simulink model "Complete_SAD_model"  (R2025b)
settings: Solver=ode4  StartTime=0.0  StopTime=10  FixedStep=0.01  RelTol=1e-3
values from neighbouring files (symbols this model uses):
  A = eye(3)    [Initial_condition.m]
  a_pink = exp(-2*pi*fc_pink*Ts_m*k_pink)    [Initial_condition.m]
  acc = deg2rad(0.5*randn)    [Initial_condition.m]
  Ap = eye(3)    [Initial_condition.m]
  D = 500*10^-12    (= 5e-10)    [Initial_condition.m]
  delay = 1    [Initial_condition.m]
  inv_Ir = inv(Ir)    [Initial_condition.m]
  Ir = diag([Irx,Iry,Irz])    [Initial_condition.m]
  J_B = diag([Ix,Iy,Iz])    [Initial_condition.m]
  m = [0.01; 0.01; 0.01]    [Initial_condition.m]
  m_max = [0.65; 0.65; 0.5]    [Initial_condition.m]
  Mr_max = [0.01; 0.01; 0.01]    [Initial_condition.m]
  mu_earth = 398600.433    [Initial_condition.m]
  mu_sun = 132712440017.987    (= 132712440018)    [Initial_condition.m]
  non_ort = deg2rad(-1+2*rand)    [Initial_condition.m]
  omega0 = [wx;wy;wz]    [Initial_condition.m]
  rES0_ECI = [0 AU 0]    [Initial_condition.m]
  seed = 0    [Initial_condition.m]
  sigma = (2*pi/60)/3    (= 0.0349065850399)    [Initial_condition.m]
  Ts_m = 1/f_m    (= 0.1)    [Initial_condition.m]
  Ts_ss = 1/f_ss    (= 0.1)    [Initial_condition.m]
  vES0_ECI = [(-sqrt(mu_sun/norm(rES0_ECI))) 0 0 ]    [Initial_condition.m]
  w_max = [250; 250; 250]    [Initial_condition.m]
undefined symbols (not defined in the file or in its folder): dspblkCoreblockFVToolHelper, gcbh, K, r0_ECI, v0_ECI
libraries: matrix_library x15, dspmathops x3, dspfdesign x3, vrlib x2
(part 3 of 3)

== matlab function Complete_SAD_model/Subsystem3/Disturbance Torques/MAGNETIC FIELD PERTURBATION1/MATLAB Function ==
  data: alfa input; delta input; r_scalar input; B_IN output; t input
function B_IN = fcn(alfa, delta, r_scalar, t)
% Magnetic field model of order 5 with g and h coefficients updated to 2025
% The output B_IN is in nT

alfa0_G = 0; % We assume the rigt ascension of Greenwich is zero at t=0
alfa_G = (2*pi/86164)*t + alfa0_G; % Right ascension of Greenwich as a function of time

%% Components of B wrt the Earth rotating fixed frame
%Br = @(psi,r,theta)1.0./r.^6.*(cos(theta).^2.*(-3.355125e+3)+cos(theta).^4.*3.9143125e+3+((sqrt(1.0e+1).*sin(theta.*2.0))./1.6e+1+sqrt(1.0e+1).*sin(theta.*4.0).*(7.0./3.2e+1)).*(cos(psi).*7.996e+2+sin(psi).*2.786e+2)+(sqrt(3.5e+1).*sin(theta).^4.*(cos(psi.*4.0).*1.2e+1-sin(psi.*4.0).*3.754e+2))./8.0-(sqrt(7.0e+1).*cos(theta).*sin(theta).^3.*(cos(psi.*3.0).*2.811e+2-sin(psi.*3.0).*2.12e+2))./4.0-(sqrt(5.0).*sin(theta).^2.*(sin(theta).^2.*7.0-6.0).*(cos(psi.*2.0).*(2.79e+2./5.0)-sin(psi.*2.0).*1.34e+2))./4.0+3.355125e+2).*3.343610149269505e+23+1.0./r.^5.*(cos(theta).*(cos(theta).^2.*5.0-3.0).*6.8045e+2+(sqrt(1.0e+1).*sin(theta).^3.*(cos(psi.*3.0).*4.534e+2-sin(psi.*3.0).*5.496e+2))./4.0+(sqrt(6.0).*sin(theta).*(sin(theta).^2.*5.0-4.0).*(cos(psi).*2.4042e+3+sin(psi).*(5.69e+2./1.0e+1)))./4.0-(sqrt(1.5e+1).*cos(theta).*(cos(psi.*2.0).*1.2438e+3+sin(psi.*2.0).*2.376e+2).*(cos(theta).^2-1.0))./2.0).*4.198537308767232e+19+1.0./r.^4.*(cos(theta).^2.*(-3.8343e+3)+(sqrt(3.0).*sin(theta).^2.*(cos(psi.*2.0).*1.6487e+3-sin(psi.*2.0).*8.142e+2))./2.0+(sqrt(3.0).*sin(theta.*2.0).*(cos(psi).*2.9509e+3-sin(psi).*3.1336e+3))./2.0+1.2781e+3).*4.942556869526643e+15+1.0./r.^7.*(sin(theta).^5.*(cos(psi.*5.0).*(2.09e+2./1.0e+1)+sin(psi.*5.0).*(5.31e+2./5.0)).*7.01560760020114e-1-cos(theta).*(cos(theta).^2.*-7.0e+1+cos(theta).^4.*6.3e+1+1.5e+1).*2.91125e+1-cos(theta).*sin(theta).^4.*(cos(psi.*4.0).*1.419e+2-sin(psi.*4.0).*(4.29e+2./1.0e+1)).*2.218529918662356+sqrt(1.5e+1).*(cos(psi).*3.69e+2+sin(psi).*(4.53e+2./1.0e+1)).*(sin(theta)-sin(theta).^3.*(7.0./2.0)+sin(theta).^5.*(2.1e+1./8.0))+(sqrt(7.0e+1).*sin(theta).^3.*(sin(theta).^2.*9.0-8.0).*(cos(psi.*3.0).*1.387e+2+sin(psi.*3.0).*1.229e+2))./1.6e+1-(sqrt(1.05e+2).*cos(theta).*(cos(psi.*2.0).*(9.36e+2./5.0)+sin(psi.*2.0).*2.2e+2).*(cos(theta).^2.*-4.0+cos(theta).^4.*3.0+1.0))./4.0).*2.556256831319522e+27-1.0./r.^3.*(cos(theta).*2.935e+4+sin(theta).*(cos(psi).*1.4103e+3-sin(psi).*4.5455e+3)).*5.17193205622e+11;
%Btheta = @(psi,r,theta)-(1.0./r.^5.*(cos(theta).*sin(theta).*6.71025e+3-cos(theta).^3.*sin(theta).*1.565725e+4+((sqrt(1.0e+1).*cos(theta.*2.0))./8.0+sqrt(1.0e+1).*cos(theta.*4.0).*(7.0./8.0)).*(cos(psi).*7.996e+2+sin(psi).*2.786e+2)+(sqrt(7.0e+1).*sin(theta).^4.*(cos(psi.*3.0).*2.811e+2-sin(psi.*3.0).*2.12e+2))./4.0-sqrt(5.0).*cos(theta).*sin(theta).^3.*(cos(psi.*2.0).*(2.79e+2./5.0)-sin(psi.*2.0).*1.34e+2).*(7.0./2.0)+(sqrt(3.5e+1).*cos(theta).*sin(theta).^3.*(cos(psi.*4.0).*1.2e+1-sin(psi.*4.0).*3.754e+2))./2.0-sqrt(7.0e+1).*cos(theta).^2.*sin(theta).^2.*(cos(psi.*3.0).*2.811e+2-sin(psi.*3.0).*2.12e+2).*(3.0./4.0)-(sqrt(5.0).*cos(theta).*sin(theta).*(sin(theta).^2.*7.0-6.0).*(cos(psi.*2.0).*(2.79e+2./5.0)-sin(psi.*2.0).*1.34e+2))./2.0).*6.687220298539009e+22+1.0./r.^4.*(sin(theta).*(cos(theta).^2.*5.0-3.0).*(-6.8045e+2)-cos(theta).^2.*sin(theta).*6.8045e+3+sqrt(1.0e+1).*cos(theta).*sin(theta).^2.*(cos(psi.*3.0).*4.534e+2-sin(psi.*3.0).*5.496e+2).*(3.0./4.0)+sqrt(1.5e+1).*cos(theta).^2.*sin(theta).*(cos(psi.*2.0).*1.2438e+3+sin(psi.*2.0).*2.376e+2)+(sqrt(6.0).*cos(theta).*(sin(theta).^2.*5.0-4.0).*(cos(psi).*2.4042e+3+sin(psi).*(5.69e+2./1.0e+1)))./4.0+sqrt(6.0).*cos(theta).*sin(theta).^2.*(cos(psi).*2.4042e+3+sin(psi).*(5.69e+2./1.0e+1)).*(5.0./2.0)+(sqrt(1.5e+1).*sin(theta).*(cos(psi.*2.0).*1.2438e+3+sin(psi.*2.0).*2.376e+2).*(cos(theta).^2-1.0))./2.0).*1.049634327191808e+19+1.0./r.^3.*(cos(theta).*sin(theta).*7.6686e+3+sqrt(3.0).*cos(theta.*2.0).*(cos(psi).*2.9509e+3-sin(psi).*3.1336e+3)+sqrt(3.0).*cos(theta).*sin(theta).*(cos(psi.*2.0).*1.6487e+3-sin(psi.*2.0).*8.142e+2)).*1.647518956508881e+15+1.0./r.^6.*(cos(theta).*(cos(theta).*sin(theta).*1.4e+2-cos(theta).^3.*sin(theta).*2.52e+2).*(-2.91125e+1)+sin(theta).^5.*(cos(psi.*4.0).*1.419e+2-sin(psi.*4.0).*(4.29e+2./1.0e+1)).*2.218529918662356+sin(theta).*(cos(theta).^2.*-7.0e+1+cos(theta).^4.*6.3e+1+1.5e+1).*2.91125e+1+cos(theta).*sin(theta).^4.*(cos(psi.*5.0).*(2.09e+2./1.0e+1)+sin(psi.*5.0).*(5.31e+2./5.0)).*3.50780380010057-cos(theta).^2.*sin(theta).^3.*(cos(psi.*4.0).*1.419e+2-sin(psi.*4.0).*(4.29e+2./1.0e+1)).*8.874119674649425+sqrt(1.5e+1).*(cos(psi).*3.69e+2+sin(psi).*(4.53e+2./1.0e+1)).*(cos(theta)-cos(theta).*sin(theta).^2.*(2.1e+1./2.0)+cos(theta).*sin(theta).^4.*(1.05e+2./8.0))-(sqrt(1.05e+2).*cos(theta).*(cos(psi.*2.0).*(9.36e+2./5.0)+sin(psi.*2.0).*2.2e+2).*(cos(theta).*sin(theta).*8.0-cos(theta).^3.*sin(theta).*1.2e+1))./4.0+sqrt(7.0e+1).*cos(theta).*sin(theta).^4.*(cos(psi.*3.0).*1.387e+2+sin(psi.*3.0).*1.229e+2).*(9.0./8.0)+(sqrt(1.05e+2).*sin(theta).*(cos(psi.*2.0).*(9.36e+2./5.0)+sin(psi.*2.0).*2.2e+2).*(cos(theta).^2.*-4.0+cos(theta).^4.*3.0+1.0))./4.0+sqrt(7.0e+1).*cos(theta).*sin(theta).^2.*(sin(theta).^2.*9.0-8.0).*(cos(psi.*3.0).*1.387e+2+sin(psi.*3.0).*1.229e+2).*(3.0./1.6e+1)).*4.260428052199203e+26+1.0./r.^2.*(sin(theta).*2.935e+4-cos(theta).*(cos(psi).*1.4103e+3-sin(psi).*4.5455e+3)).*2.58596602811e+11)./r;
%Bpsi = @(psi,r,theta)-(1.0./r.^3.*((sqrt(3.0).*sin(theta).^2.*(cos(psi.*2.0).*1.6284e+3+sin(psi.*2.0).*3.2974e+3))./2.0+(sqrt(3.0).*sin(theta.*2.0).*(cos(psi).*3.1336e+3+sin(psi).*2.9509e+3))./2.0).*-1.647518956508881e+15-1.0./r.^4.*((sqrt(1.0e+1).*sin(theta).^3.*(cos(psi.*3.0).*1.6488e+3+sin(psi.*3.0).*1.3602e+3))./4.0-(sqrt(6.0).*sin(theta).*(sin(theta).^2.*5.0-4.0).*(cos(psi).*(5.69e+2./1.0e+1)-sin(psi).*2.4042e+3))./4.0+(sqrt(1.5e+1).*cos(theta).*(cos(psi.*2.0).*4.752e+2-sin(psi.*2.0).*2.4876e+3).*(cos(theta).^2-1.0))./2.0).*1.049634327191808e+19+1.0./r.^5.*(((sqrt(1.0e+1).*sin(theta.*2.0))./1.6e+1+sqrt(1.0e+1).*sin(theta.*4.0).*(7.0./3.2e+1)).*(cos(psi).*2.786e+2-sin(psi).*7.996e+2)-(sqrt(3.5e+1).*sin(theta).^4.*(cos(psi.*4.0).*1.5016e+3+sin(psi.*4.0).*4.8e+1))./8.0+(sqrt(7.0e+1).*cos(theta).*sin(theta).^3.*(cos(psi.*3.0).*6.36e+2+sin(psi.*3.0).*8.433e+2))./4.0+(sqrt(5.0).*sin(theta).^2.*(sin(theta).^2.*7.0-6.0).*(cos(psi.*2.0).*2.68e+2+sin(psi.*2.0).*(5.58e+2./5.0)))./4.0).*6.687220298539009e+22+1.0./r.^6.*(sin(theta).^5.*(cos(psi.*5.0).*5.31e+2-sin(psi.*5.0).*(2.09e+2./2.0)).*7.01560760020114e-1+cos(theta).*sin(theta).^4.*(cos(psi.*4.0).*(8.58e+2./5.0)+sin(psi.*4.0).*5.676e+2).*2.218529918662356+sqrt(1.5e+1).*(cos(psi).*(4.53e+2./1.0e+1)-sin(psi).*3.69e+2).*(sin(theta)-sin(theta).^3.*(7.0./2.0)+sin(theta).^5.*(2.1e+1./8.0))+(sqrt(7.0e+1).*sin(theta).^3.*(sin(theta).^2.*9.0-8.0).*(cos(psi.*3.0).*3.687e+2-sin(psi.*3.0).*4.161e+2))./1.6e+1-(sqrt(1.05e+2).*cos(theta).*(cos(psi.*2.0).*4.4e+2-sin(psi.*2.0).*3.744e+2).*(cos(theta).^2.*-4.0+cos(theta).^4.*3.0+1.0))./4.0).*4.260428052199203e+26+1.0./r.^2.*sin(theta).*(cos(psi).*4.5455e+3+sin(psi).*1.4103e+3).*2.58596602811e+11)./(r.*sin(theta));
Br = @(psi,r,theta)1.0./r.^6.*(cos(theta).^2.*(-3.355125e+3)+cos(theta).^4.*3.9143125e+3+((sqrt(1.0e+1).*sin(theta.*2.0))./1.6e+1+sqrt(1.0e+1).*sin(theta.*4.0).*(7.0./3.2e+1)).*(cos(psi).*7.996e+2+sin(psi).*2.786e+2)+(sqrt(3.5e+1).*sin(theta).^4.*(cos(psi.*4.0).*1.2e+1-sin(psi.*4.0).*3.754e+2))./8.0-(sqrt(7.0e+1).*cos(theta).*sin(theta).^3.*(cos(psi.*3.0).*2.811e+2-sin(psi.*3.0).*2.12e+2))./4.0-(sqrt(5.0).*sin(theta).^2.*(sin(theta).^2.*7.0-6.0).*(cos(psi.*2.0).*(2.79e+2./5.0)-sin(psi.*2.0).*1.34e+2))./4.0+3.355125e+2).*3.343610149269505e+23+1.0./r.^8.*(cos(theta).^2.*4.2196875e+2-cos(theta).^4.*1.26590625e+3+cos(theta).^6.*9.2833125e+2-sin(theta).^6.*(cos(psi.*6.0).*(3.04e+2./5.0)-sin(psi.*6.0).*(3.64e+2./5.0)).*6.716932893813961e-1+(cos(psi).*(3.19e+2./5.0)-sin(psi).*(9.2e+1./5.0)).*(sqrt(2.1e+1).*sin(theta.*2.0).*(5.0./2.56e+2)+sqrt(2.1e+1).*sin(theta.*4.0).*(3.0./6.4e+1)+sqrt(2.1e+1).*sin(theta.*6.0).*(3.3e+1./2.56e+2))+cos(theta).*sin(theta).^5.*(cos(psi.*5.0).*(1.49e+2./1.0e+1)+sin(psi.*5.0).*(1.09e+2./1.0e+1)).*2.326813808623286+sin(theta).^4.*(sin(theta).^2.*1.1e+1-1.0e+1).*(cos(psi.*4.0).*(4.09e+2./1.0e+1)+sin(psi.*4.0).*(2.99e+2./5.0)).*4.960783708246107e-1+(sqrt(2.1e+2).*sin(theta).^2.*(cos(psi.*2.0).*(7.67e+2./1.0e+1)+sin(psi.*2.0).*(8.4e+1./5.0)).*(sin(theta).^2.*-4.8e+1+sin(theta).^4.*3.3e+1+1.6e+1))./3.2e+1-(sqrt(2.1e+2).*cos(theta).*sin(theta).^3.*(cos(psi.*3.0).*1.157e+2-sin(psi.*3.0).*(4.89e+2./1.0e+1)).*(cos(theta).^2.*1.1e+1-3.0))./1.6e+1-6.43e+2./3.2e+1).*1.900023098439278e+31+1.0./r.^10.*((cos(psi).*(1.09e+2./1.0e+1)+sin(psi).*(3.6e+1./5.0)).*(sin(theta.*2.0).*5.126953125e-2+sin(theta.*4.0).*1.1279296875e-1+sin(theta.*6.0).*2.0947265625e-1+sin(theta.*8.0).*5.23681640625e-1)-cos(theta).^2.*2.27390625e+2+cos(theta).^4.*1.2506484375e+3-cos(theta).^6.*2.167790625e+3+cos(theta).^8.*1.16131640625e+3+sin(theta).^8.*(cos(psi.*8.0)+sin(psi.*8.0).*(3.9e+1./1.0e+1)).*6.267066542400439e-1-cos(theta).*sin(theta).^7.*(cos(psi.*7.0).*(8.4e+1./5.0)+sin(psi.*7.0).*(2.6e+1./5.0)).*2.506826616960176-sin(theta).^6.*(sin(theta).^2.*1.5e+1-1.4e+1).*(cos(psi.*6.0).*(1.49e+2./1.0e+1)+sin(psi.*6.0).*(7.0./1.0e+1)).*4.576818286211503e-1-sin(theta).^4.*(cos(psi.*4.0).*(1.09e+2./5.0)+sin(psi.*4.0).*(9.7e+1./1.0e+1)).*(sin(theta).^2.*-1.04e+2+sin(theta).^4.*6.5e+1+4.0e+1).*4.113264556590057e-1+cos(theta).*sin(theta).^5.*(cos(psi.*5.0).*(1.69e+2./1.0e+1)+sin(psi.*5.0).*(1.27e+2./1.0e+1)).*(cos(theta).^2.*5.0-1.0).*2.96611725366682+cos(theta).*sin(theta).^3.*(cos(psi.*3.0).*2.0+sin(psi.*3.0).*(2.3e+1./2.0)).*(cos(theta).^2.*-2.6e+1+cos(theta).^4.*3.9e+1+3.0).*1.062040341747902+sqrt(7.0e+1).*sin(theta).^2.*(cos(psi.*2.0).*(3.5e+1./2.0)+sin(psi.*2.0).*(6.3e+1./5.0)).*(sin(theta).^2.*1.76e+2-sin(theta).^4.*2.86e+2+sin(theta).^6.*1.43e+2-3.2e+1).*4.6875e-2+6.31640625).*9.915589987374597e+38-1.0./r.^11.*(sin(theta).^9.*(cos(psi.*9.0).*(6.4e+1./5.0)-sin(psi.*9.0).*(4.9e+1./5.0)).*6.090493921755238e-1-cos(theta).*(cos(theta).^2.*-4.62e+3+cos(theta).^4.*1.8018e+4-cos(theta).^6.*2.574e+4+cos(theta).^8.*1.2155e+4+3.15e+2).*3.671875e-2+cos(theta).*sin(theta).^8.*(cos(psi.*8.0).*(8.7e+1./1.0e+1)-sin(psi.*8.0).*(4.0./5.0)).*2.583977731709148+sin(theta).^7.*(sin(theta).^2.*1.7e+1-1.6e+1).*(cos(psi.*7.0).*(4.3e+1./5.0)-sin(psi.*7.0).*(3.0./5.0)).*4.431485250278681e-1-sin(theta).^3.*(cos(psi.*3.0)./5.0-sin(psi.*3.0).*(8.3e+1./1.0e+1)).*(sin(theta).^2.*3.12e+2-sin(theta).^4.*4.68e+2+sin(theta).^6.*2.21e+2-6.4e+1).*3.754879637718099e-1+sin(theta).^5.*(cos(psi.*5.0).*(1.31e+2./1.0e+1)+sin(psi.*5.0).*(5.3e+1./1.0e+1)).*(sin(theta).^2.*-1.4e+2+sin(theta).^4.*8.5e+1+5.6e+1).*3.96364090436432e-1-cos(theta).*sin(theta).^6.*(cos(psi.*6.0).*(1.2e+1./5.0)+sin(psi.*6.0).*(3.6e+1./5.0)).*(cos(theta).^2.*1.7e+1-3.0).*1.023407680863301-sqrt(5.0).*sin(theta).*(cos(psi).*8.0-sin(psi).*(1.24e+2./5.0)).*(sin(theta).^2.*-1.408e+3+sin(theta).^4.*4.576e+3-sin(theta).^6.*5.72e+3+sin(theta).^8.*2.431e+3+1.28e+2).*2.34375e-2+cos(theta).*sin(theta).^4.*(cos(psi.*4.0).*(5.0./2.0)+sin(psi.*4.0).*(1.7e+1./5.0)).*(cos(theta).^2.*-1.0e+1+cos(theta).^4.*1.7e+1+1.0).*3.316219904216999+sqrt(1.1e+2).*cos(theta).*(cos(psi.*2.0).*3.0+sin(psi.*2.0).*(1.21e+2./1.0e+1)).*(cos(theta).^2.*-9.8e+1+cos(theta).^4.*3.64e+2-cos(theta).^6.*4.94e+2+cos(theta).^8.*2.21e+2+7.0).*4.6875e-2).*7.019135978840395e+42+1.0./r.^5.*(cos(theta).*(cos(theta).^2.*5.0-3.0).*6.8045e+2+(sqrt(1.0e+1).*sin(theta).^3.*(cos(psi.*3.0).*4.534e+2-sin(psi.*3.0).*5.496e+2))./4.0+(sqrt(6.0).*sin(theta).*(sin(theta).^2.*5.0-4.0).*(cos(psi).*2.4042e+3+sin(psi).*(5.69e+2./1.0e+1)))./4.0-(sqrt(1.5e+1).*cos(theta).*(cos(psi.*2.0).*1.2438e+3+sin(psi.*2.0).*2.376e+2).*(cos(theta).^2-1.0))./2.0).*4.198537308767232e+19+1.0./r.^4.*(cos(theta).^2.*(-3.8343e+3)+(sqrt(3.0).*sin(theta).^2.*(cos(psi.*2.0).*1.6487e+3-sin(psi.*2.0).*8.142e+2))./2.0+(sqrt(3.0).*sin(theta.*2.0).*(cos(psi).*2.9509e+3-sin(psi).*3.1336e+3))./2.0+1.2781e+3).*4.942556869526643e+15+1.0./r.^9.*(sin(theta).^7.*(cos(psi.*7.0).*(1.43e+2./1.0e+1)-sin(psi.*7.0).*(1.1e+1./5.0)).*6.472598492877493e-1+cos(theta).*(cos(theta).^2.*3.15e+2-cos(theta).^4.*6.93e+2+cos(theta).^6.*4.29e+2-3.5e+1).*4.975-cos(theta).*sin(theta).^6.*(cos(psi.*6.0).*(5.6e+1./5.0)+sin(psi.*6.0).*(2.51e+2./1.0e+1)).*2.421824596249695-sin(theta).^5.*(sin(theta).^2.*1.3e+1-1.2e+1).*(cos(psi.*5.0).*(5.0./2.0)-sin(psi.*5.0).*(3.7e+1./5.0)).*4.749588797990833e-1+cos(theta).*sin(theta).^4.*(cos(psi.*4.0).*(7.9e+1./5.0)+sin(psi.*4.0).*(4.7e+1./2.0)).*(cos(theta).^2.*1.3e+1-3.0).*9.499177595981665e-1+sqrt(2.1e+1).*sin(theta).^3.*(cos(psi.*3.0).*(5.93e+2./1.0e+1)-sin(psi.*3.0)).*(sin(theta).^2.*-2.2e+2+sin(theta).^4.*1.43e+2+8.0e+1).*3.125e-2+sqrt(4.2e+1).*cos(theta).*(cos(psi.*2.0).*(4.4e+1./5.0)+sin(psi.*2.0).*(7.2e+1./5.0)).*(cos(theta).^2.*1.25e+2-cos(theta).^4.*2.53e+2+cos(theta).^6.*1.43e+2-1.5e+1).*3.125e-2+sqrt(7.0).*sin(theta).*(cos(psi).*(7.69e+2./1.0e+1)+sin(psi).*(4.89e+2./1.0e+1)).*(sin(theta).^2.*4.32e+2-sin(theta).^4.*7.92e+2+sin(theta).^6.*4.29e+2-6.4e+1).*3.125e-2).*1.383433961160759e+35+1.0./r.^7.*(sin(theta).^5.*(cos(psi.*5.0).*(2.09e+2./1.0e+1)+sin(psi.*5.0).*(5.31e+2./5.0)).*7.01560760020114e-1-cos(theta).*(cos(theta).^2.*-7.0e+1+cos(theta).^4.*6.3e+1+1.5e+1).*2.91125e+1-cos(theta).*sin(theta).^4.*(cos(psi.*4.0).*1.419e+2-sin(psi.*4.0).*(4.29e+2./1.0e+1)).*2.218529918662356+sqrt(1.5e+1).*(cos(psi).*3.69e+2+sin(psi).*(4.53e+2./1.0e+1)).*(sin(theta)-sin(theta).^3.*(7.0./2.0)+sin(theta).^5.*(2.1e+1./8.0))+(sqrt(7.0e+1).*sin(theta).^3.*(sin(theta).^2.*9.0-8.0).*(cos(psi.*3.0).*1.387e+2+sin(psi.*3.0).*1.229e+2))./1.6e+1-(sqrt(1.05e+2).*cos(theta).*(cos(psi.*2.0).*(9.36e+2./5.0)+sin(psi.*2.0).*2.2e+2).*(cos(theta).^2.*-4.0+cos(theta).^4.*3.0+1.0))./4.0).*2.556256831319522e+27-1.0./r.^12.*(cos(theta).^2.*1.7595703125e+1-cos(theta).^4.*1.5249609375e+2+cos(theta).^6.*4.5748828125e+2-cos(theta).^8.*5.55521484375e+2+cos(theta).^10.*2.34553515625e+2+sin(theta).^10.*(cos(psi.*1.0e+1).*(3.9e+1./1.0e+1)+sin(psi.*1.0e+1).*9.0).*5.936279171365732e-1+cos(theta).*sin(theta).^9.*(cos(psi.*9.0).*(1.3e+1./5.0)-sin(psi.*9.0).*(9.0./1.0e+1)).*2.65478475211798-sin(theta).^4.*(cos(psi.*4.0)-sin(psi.*4.0).*(2.7e+1./5.0)).*(sin(theta).^2.*5.04e+2-sin(theta).^4.*7.14e+2+sin(theta).^6.*3.23e+2-1.12e+2).*3.618292555284191e-1+sin(theta).^8.*(sin(theta).^2.*1.9e+1-1.8e+1).*(cos(psi.*8.0).*(9.0./1.0e+1)-sin(psi.*8.0).*(1.9e+1./5.0)).*4.306629552848578e-1+sin(theta).^6.*(cos(psi.*6.0).*(9.0./1.0e+1)-sin(psi.*6.0).*(2.0./5.0)).*(sin(theta).^2.*-5.44e+2+sin(theta).^4.*3.23e+2+2.24e+2).*1.279259601079126e-1-cos(theta).*sin(theta).^7.*(cos(psi.*7.0).*(3.0./2.0)-sin(psi.*7.0).*(2.1e+1./5.0)).*(cos(theta).^2.*1.9e+1-3.0).*1.05490449156695-cos(theta).*sin(theta).^3.*(cos(psi.*3.0).*2.0+sin(psi.*3.0).*(5.0./2.0)).*(cos(theta).^2.*1.05e+2-cos(theta).^4.*3.57e+2+cos(theta).^6.*3.23e+2-7.0).*5.117038404316505e-1-sqrt(1.65e+2).*sin(theta).^2.*(cos(psi.*2.0)./5.0+sin(psi.*2.0)./1.0e+1).*(sin(theta).^2.*-3.328e+3+sin(theta).^4.*9.36e+3-sin(theta).^6.*1.0608e+4+sin(theta).^8.*4.199e+3+3.84e+2).*3.90625e-3+cos(theta).*sin(theta).^5.*(cos(psi.*5.0)./2.0+sin(psi.*5.0).*9.0).*(cos(theta).^2.*-1.7e+2+cos(theta).^4.*3.23e+2+1.5e+1).*2.288409143105751e-1+sqrt(5.5e+1).*cos(theta).*sin(theta).*(cos(psi).*(3.2e+1./5.0)-sin(psi).*(3.3e+1./1.0e+1)).*(cos(theta).^2.*-1.092e+3+cos(theta).^4.*4.914e+3-cos(theta).^6.*7.956e+3+cos(theta).^8.*4.199e+3+6.3e+1).*7.812499999999999e-3-3.19921875e-1).*4.919080685331137e+46-1.0./r.^3.*(cos(theta).*2.935e+4+sin(theta).*(cos(psi).*1.4103e+3-sin(psi).*4.5455e+3)).*5.17193205622e+11;
Btheta = @(psi,r,theta)-(1.0./r.^8.*(sin(theta).^7.*(cos(psi.*6.0).*(5.6e+1./5.0)+sin(psi.*6.0).*(2.51e+2./1.0e+1)).*(-2.421824596249695)+sin(theta).*(cos(theta).^2.*3.15e+2-cos(theta).^4.*6.93e+2+cos(theta).^6.*4.29e+2-3.5e+1).*4.975+cos(theta).*(cos(theta).*sin(theta).*6.3e+2-cos(theta).^3.*sin(theta).*2.772e+3+cos(theta).^5.*sin(theta).*2.574e+3).*4.975+cos(theta).*sin(theta).^6.*(cos(psi.*5.0).*(5.0./2.0)-sin(psi.*5.0).*(3.7e+1./5.0)).*1.234893087477616e+1-cos(theta).*sin(theta).^6.*(cos(psi.*7.0).*(1.43e+2./1.0e+1)-sin(psi.*7.0).*(1.1e+1./5.0)).*4.530818945014245+sin(theta).^5.*(cos(psi.*4.0).*(7.9e+1./5.0)+sin(psi.*4.0).*(4.7e+1./2.0)).*(cos(theta).^2.*1.3e+1-3.0).*9.499177595981665e-1+cos(theta).^2.*sin(theta).^5.*(cos(psi.*4.0).*(7.9e+1./5.0)+sin(psi.*4.0).*(4.7e+1./2.0)).*2.469786174955233e+1+cos(theta).^2.*sin(theta).^5.*(cos(psi.*6.0).*(5.6e+1./5.0)+sin(psi.*6.0).*(2.51e+2./1.0e+1)).*1.453094757749817e+1+cos(theta).*sin(theta).^4.*(sin(theta).^2.*1.3e+1-1.2e+1).*(cos(psi.*5.0).*(5.0./2.0)-sin(psi.*5.0).*(3.7e+1./5.0)).*2.374794398995416+sqrt(4.2e+1).*sin(theta).*(cos(psi.*2.0).*(4.4e+1./5.0)+sin(psi.*2.0).*(7.2e+1./5.0)).*(cos(theta).^2.*1.25e+2-cos(theta).^4.*2.53e+2+cos(theta).^6.*1.43e+2-1.5e+1).*3.125e-2-cos(theta).^2.*sin(theta).^3.*(cos(psi.*4.0).*(7.9e+1./5.0)+sin(psi.*4.0).*(4.7e+1./2.0)).*(cos(theta).^2.*1.3e+1-3.0).*3.799671038392666+sqrt(2.1e+1).*sin(theta).^3.*(cos(psi.*3.0).*(5.93e+2./1.0e+1)-sin(psi.*3.0)).*(cos(theta).*sin(theta).*4.4e+2-cos(theta).*sin(theta).^3.*5.72e+2).*3.125e-2+sqrt(4.2e+1).*cos(theta).*(cos(psi.*2.0).*(4.4e+1./5.0)+sin(psi.*2.0).*(7.2e+1./5.0)).*(cos(theta).*sin(theta).*2.5e+2-cos(theta).^3.*sin(theta).*1.012e+3+cos(theta).^5.*sin(theta).*8.58e+2).*3.125e-2-sqrt(7.0).*cos(theta).*(cos(psi).*(7.69e+2./1.0e+1)+sin(psi).*(4.89e+2./1.0e+1)).*(sin(theta).^2.*4.32e+2-sin(theta).^4.*7.92e+2+sin(theta).^6.*4.29e+2-6.4e+1).*3.125e-2-sqrt(7.0).*sin(theta).*(cos(psi).*(7.69e+2./1.0e+1)+sin(psi).*(4.89e+2./1.0e+1)).*(cos(theta).*sin(theta).*8.64e+2-cos(theta).*sin(theta).^3.*3.168e+3+cos(theta).*sin(theta).^5.*2.574e+3).*3.125e-2-sqrt(2.1e+1).*cos(theta).*sin(theta).^2.*(cos(psi.*3.0).*(5.93e+2./1.0e+1)-sin(psi.*3.0)).*(sin(theta).^2.*-2.2e+2+sin(theta).^4.*1.43e+2+8.0e+1).*9.375e-2).*-1.729292451450949e+34+1.0./r.^5.*(cos(theta).*sin(theta).*6.71025e+3-cos(theta).^3.*sin(theta).*1.565725e+4+((sqrt(1.0e+1).*cos(theta.*2.0))./8.0+sqrt(1.0e+1).*cos(theta.*4.0).*(7.0./8.0)).*(cos(psi).*7.996e+2+sin(psi).*2.786e+2)+(sqrt(7.0e+1).*sin(theta).^4.*(cos(psi.*3.0).*2.811e+2-sin(psi.*3.0).*2.12e+2))./4.0-sqrt(5.0).*cos(theta).*sin(theta).^3.*(cos(psi.*2.0).*(2.79e+2./5.0)-sin(psi.*2.0).*1.34e+2).*(7.0./2.0)+(sqrt(3.5e+1).*cos(theta).*sin(theta).^3.*(cos(psi.*4.0).*1.2e+1-sin(psi.*4.0).*3.754e+2))./2.0-sqrt(7.0e+1).*cos(theta).^2.*sin(theta).^2.*(cos(psi.*3.0).*2.811e+2-sin(psi.*3.0).*2.12e+2).*(3.0./4.0)-(sqrt(5.0).*cos(theta).*sin(theta).*(sin(theta).^2.*7.0-6.0).*(cos(psi.*2.0).*(2.79e+2./5.0)-sin(psi.*2.0).*1.34e+2))./2.0).*6.687220298539009e+22+1.0./r.^4.*(sin(theta).*(cos(theta).^2.*5.0-3.0).*(-6.8045e+2)-cos(theta).^2.*sin(theta).*6.8045e+3+sqrt(1.0e+1).*cos(theta).*sin(theta).^2.*(cos(psi.*3.0).*4.534e+2-sin(psi.*3.0).*5.496e+2).*(3.0./4.0)+sqrt(1.5e+1).*cos(theta).^2.*sin(theta).*(cos(psi.*2.0).*1.2438e+3+sin(psi.*2.0).*2.376e+2)+(sqrt(6.0).*cos(theta).*(sin(theta).^2.*5.0-4.0).*(cos(psi).*2.4042e+3+sin(psi).*(5.69e+2./1.0e+1)))./4.0+sqrt(6.0).*cos(theta).*sin(theta).^2.*(cos(psi).*2.4042e+3+sin(psi).*(5.69e+2./1.0e+1)).*(5.0./2.0)+(sqrt(1.5e+1).*sin(theta).*(cos(psi.*2.0).*1.2438e+3+sin(psi.*2.0).*2.376e+2).*(cos(theta).^2-1.0))./2.0).*1.049634327191808e+19-1.0./r.^10.*(sin(theta).*(cos(theta).^2.*-4.62e+3+cos(theta).^4.*1.8018e+4-cos(theta).^6.*2.574e+4+cos(theta).^8.*1.2155e+4+3.15e+2).*3.671875e-2-cos(theta).*(cos(theta).*sin(theta).*9.24e+3-cos(theta).^3.*sin(theta).*7.2072e+4+cos(theta).^5.*sin(theta).*1.5444e+5-cos(theta).^7.*sin(theta).*9.724e+4).*3.671875e-2-sin(theta).^9.*(cos(psi.*8.0).*(8.7e+1./1.0e+1)-sin(psi.*8.0).*(4.0./5.0)).*2.583977731709148+cos(theta).*sin(theta).^8.*(cos(psi.*7.0).*(4.3e+1./5.0)-sin(psi.*7.0).*(3.0./5.0)).*1.506704985094751e+1+cos(theta).*sin(theta).^8.*(cos(psi.*9.0).*(6.4e+1./5.0)-sin(psi.*9.0).*(4.9e+1./5.0)).*5.481444529579714+sin(theta).^7.*(cos(psi.*6.0).*(1.2e+1./5.0)+sin(psi.*6.0).*(3.6e+1./5.0)).*(cos(theta).^2.*1.7e+1-3.0).*1.023407680863301-sin(theta).^5.*(cos(psi.*5.0).*(1.31e+2./1.0e+1)+sin(psi.*5.0).*(5.3e+1./1.0e+1)).*(cos(theta).*sin(theta).*2.8e+2-cos(theta).*sin(theta).^3.*3.4e+2).*3.96364090436432e-1+cos(theta).^2.*sin(theta).^7.*(cos(psi.*6.0).*(1.2e+1./5.0)+sin(psi.*6.0).*(3.6e+1./5.0)).*3.479586114935223e+1+cos(theta).^2.*sin(theta).^7.*(cos(psi.*8.0).*(8.7e+1./1.0e+1)-sin(psi.*8.0).*(4.0./5.0)).*2.067182185367318e+1-sin(theta).^3.*(cos(psi.*3.0)./5.0-sin(psi.*3.0).*(8.3e+1./1.0e+1)).*(cos(theta).*sin(theta).*6.24e+2-cos(theta).*sin(theta).^3.*1.872e+3+cos(theta).*sin(theta).^5.*1.326e+3).*3.754879637718099e-1-sin(theta).^5.*(cos(psi.*4.0).*(5.0./2.0)+sin(psi.*4.0).*(1.7e+1./5.0)).*(cos(theta).^2.*-1.0e+1+cos(theta).^4.*1.7e+1+1.0).*3.316219904216999+cos(theta).*sin(theta).^4.*(cos(psi.*4.0).*(5.0./2.0)+sin(psi.*4.0).*(1.7e+1./5.0)).*(cos(theta).*sin(theta).*2.0e+1-cos(theta).^3.*sin(theta).*6.8e+1).*3.316219904216999+cos(theta).*sin(theta).^6.*(sin(theta).^2.*1.7e+1-1.6e+1).*(cos(psi.*7.0).*(4.3e+1./5.0)-sin(psi.*7.0).*(3.0./5.0)).*3.102039675195077+sqrt(1.1e+2).*cos(theta).*(cos(psi.*2.0).*3.0+sin(psi.*2.0).*(1.21e+2./1.0e+1)).*(cos(theta).*sin(theta).*1.96e+2-cos(theta).^3.*sin(theta).*1.456e+3+cos(theta).^5.*sin(theta).*2.964e+3-cos(theta).^7.*sin(theta).*1.768e+3).*4.6875e-2-cos(theta).*sin(theta).^2.*(cos(psi.*3.0)./5.0-sin(psi.*3.0).*(8.3e+1./1.0e+1)).*(sin(theta).^2.*3.12e+2-sin(theta).^4.*4.68e+2+sin(theta).^6.*2.21e+2-6.4e+1).*1.12646389131543-sqrt(5.0).*cos(theta).*(cos(psi).*8.0-sin(psi).*(1.24e+2./5.0)).*(sin(theta).^2.*-1.408e+3+sin(theta).^4.*4.576e+3-sin(theta).^6.*5.72e+3+sin(theta).^8.*2.431e+3+1.28e+2).*2.34375e-2-cos(theta).^2.*sin(theta).^5.*(cos(psi.*6.0).*(1.2e+1./5.0)+sin(psi.*6.0).*(3.6e+1./5.0)).*(cos(theta).^2.*1.7e+1-3.0).*6.140446085179805+sqrt(5.0).*sin(theta).*(cos(psi).*8.0-sin(psi).*(1.24e+2./5.0)).*(cos(theta).*sin(theta).*2.816e+3-cos(theta).*sin(theta).^3.*1.8304e+4+cos(theta).*sin(theta).^5.*3.432e+4-cos(theta).*sin(theta).^7.*1.9448e+4).*2.34375e-2+cos(theta).*sin(theta).^4.*(cos(psi.*5.0).*(1.31e+2./1.0e+1)+sin(psi.*5.0).*(5.3e+1./1.0e+1)).*(sin(theta).^2.*-1.4e+2+sin(theta).^4.*8.5e+1+5.6e+1).*1.98182045218216-sqrt(1.1e+2).*sin(theta).*(cos(psi.*2.0).*3.0+sin(psi.*2.0).*(1.21e+2./1.0e+1)).*(cos(theta).^2.*-9.8e+1+cos(theta).^4.*3.64e+2-cos(theta).^6.*4.94e+2+cos(theta).^8.*2.21e+2+7.0).*4.6875e-2+cos(theta).^2.*sin(theta).^3.*(cos(psi.*4.0).*(5.0./2.0)+sin(psi.*4.0).*(1.7e+1./5.0)).*(cos(theta).^2.*-1.0e+1+cos(theta).^4.*1.7e+1+1.0).*1.3264879616868e+1).*7.019135978840395e+41+1.0./r.^3.*(cos(theta).*sin(theta).*7.6686e+3+sqrt(3.0).*cos(theta.*2.0).*(cos(psi).*2.9509e+3-sin(psi).*3.1336e+3)+sqrt(3.0).*cos(theta).*sin(theta).*(cos(psi.*2.0).*1.6487e+3-sin(psi.*2.0).*8.142e+2)).*1.647518956508881e+15+1.0./r.^9.*(cos(theta).*sin(theta).*4.5478125e+2+sin(theta).^8.*(cos(psi.*7.0).*(8.4e+1./5.0)+sin(psi.*7.0).*(2.6e+1./5.0)).*2.506826616960176-cos(theta).^3.*sin(theta).*5.00259375e+3+cos(theta).^5.*sin(theta).*1.300674375e+4-cos(theta).^7.*sin(theta).*9.29053125e+3+(cos(psi).*(1.09e+2./1.0e+1)+sin(psi).*(3.6e+1./5.0)).*(cos(theta.*2.0).*1.025390625e-1+cos(theta.*4.0).*4.51171875e-1+cos(theta.*6.0).*1.2568359375+cos(theta.*8.0).*4.189453125)-cos(theta).*sin(theta).^7.*(cos(psi.*6.0).*(1.49e+2./1.0e+1)+sin(psi.*6.0).*(7.0./1.0e+1)).*1.373045485863451e+1-sin(theta).^6.*(cos(psi.*5.0).*(1.69e+2./1.0e+1)+sin(psi.*5.0).*(1.27e+2./1.0e+1)).*(cos(theta).^2.*5.0-1.0).*2.96611725366682+sin(theta).^4.*(cos(psi.*4.0).*(1.09e+2./5.0)+sin(psi.*4.0).*(9.7e+1./1.0e+1)).*(cos(theta).*sin(theta).*2.08e+2-cos(theta).*sin(theta).^3.*2.6e+2).*4.113264556590057e-1-cos(theta).^2.*sin(theta).^6.*(cos(psi.*7.0).*(8.4e+1./5.0)+sin(psi.*7.0).*(2.6e+1./5.0)).*1.754778631872123e+1-cos(theta).^2.*sin(theta).^6.*(cos(psi.*5.0).*(1.69e+2./1.0e+1)+sin(psi.*5.0).*(1.27e+2./1.0e+1)).*2.96611725366682e+1+cos(theta).*sin(theta).^7.*(cos(psi.*8.0)+sin(psi.*8.0).*(3.9e+1./1.0e+1)).*5.013653233920351-sin(theta).^4.*(cos(psi.*3.0).*2.0+sin(psi.*3.0).*(2.3e+1./2.0)).*(cos(theta).^2.*-2.6e+1+cos(theta).^4.*3.9e+1+3.0).*1.062040341747902+cos(theta).*sin(theta).^3.*(cos(psi.*3.0).*2.0+sin(psi.*3.0).*(2.3e+1./2.0)).*(cos(theta).*sin(theta).*5.2e+1-cos(theta).^3.*sin(theta).*1.56e+2).*1.062040341747902+sqrt(7.0e+1).*sin(theta).^2.*(cos(psi.*2.0).*(3.5e+1./2.0)+sin(psi.*2.0).*(6.3e+1./5.0)).*(cos(theta).*sin(theta).*3.52e+2-cos(theta).*sin(theta).^3.*1.144e+3+cos(theta).*sin(theta).^5.*8.58e+2).*4.6875e-2-cos(theta).*sin(theta).^5.*(sin(theta).^2.*1.5e+1-1.4e+1).*(cos(psi.*6.0).*(1.49e+2./1.0e+1)+sin(psi.*6.0).*(7.0./1.0e+1)).*2.746090971726902+cos(theta).^2.*sin(theta).^4.*(cos(psi.*5.0).*(1.69e+2./1.0e+1)+sin(psi.*5.0).*(1.27e+2./1.0e+1)).*(cos(theta).^2.*5.0-1.0).*1.48305862683341e+1-cos(theta).*sin(theta).^3.*(cos(psi.*4.0).*(1.09e+2./5.0)+sin(psi.*4.0).*(9.7e+1./1.0e+1)).*(sin(theta).^2.*-1.04e+2+sin(theta).^4.*6.5e+1+4.0e+1).*1.645305822636023+cos(theta).^2.*sin(theta).^2.*(cos(psi.*3.0).*2.0+sin(psi.*3.0).*(2.3e+1./2.0)).*(cos(theta).^2.*-2.6e+1+cos(theta).^4.*3.9e+1+3.0).*3.186121025243705+sqrt(7.0e+1).*cos(theta).*sin(theta).*(cos(psi.*2.0).*(3.5e+1./2.0)+sin(psi.*2.0).*(6.3e+1./5.0)).*(sin(theta).^2.*1.76e+2-sin(theta).^4.*2.86e+2+sin(theta).^6.*1.43e+2-3.2e+1).*9.375e-2).*1.1017322208194e+38+1.0./r.^6.*(cos(theta).*(cos(theta).*sin(theta).*1.4e+2-cos(theta).^3.*sin(theta).*2.52e+2).*(-2.91125e+1)+sin(theta).^5.*(cos(psi.*4.0).*1.419e+2-sin(psi.*4.0).*(4.29e+2./1.0e+1)).*2.218529918662356+sin(theta).*(cos(theta).^2.*-7.0e+1+cos(theta).^4.*6.3e+1+1.5e+1).*2.91125e+1+cos(theta).*sin(theta).^4.*(cos(psi.*5.0).*(2.09e+2./1.0e+1)+sin(psi.*5.0).*(5.31e+2./5.0)).*3.50780380010057-cos(theta).^2.*sin(theta).^3.*(cos(psi.*4.0).*1.419e+2-sin(psi.*4.0).*(4.29e+2./1.0e+1)).*8.874119674649425+sqrt(1.5e+1).*(cos(psi).*3.69e+2+sin(psi).*(4.53e+2./1.0e+1)).*(cos(theta)-cos(theta).*sin(theta).^2.*(2.1e+1./2.0)+cos(theta).*sin(theta).^4.*(1.05e+2./8.0))-(sqrt(1.05e+2).*cos(theta).*(cos(psi.*2.0).*(9.36e+2./5.0)+sin(psi.*2.0).*2.2e+2).*(cos(theta).*sin(theta).*8.0-cos(theta).^3.*sin(theta).*1.2e+1))./4.0+sqrt(7.0e+1).*cos(theta).*sin(theta).^4.*(cos(psi.*3.0).*1.387e+2+sin(psi.*3.0).*1.229e+2).*(9.0./8.0)+(sqrt(1.05e+2).*sin(theta).*(cos(psi.*2.0).*(9.36e+2./5.0)+sin(psi.*2.0).*2.2e+2).*(cos(theta).^2.*-4.0+cos(theta).^4.*3.0+1.0))./4.0+sqrt(7.0e+1).*cos(theta).*sin(theta).^2.*(sin(theta).^2.*9.0-8.0).*(cos(psi.*3.0).*1.387e+2+sin(psi.*3.0).*1.229e+2).*(3.0./1.6e+1)).*4.260428052199203e+26+1.0./r.^7.*(cos(theta).*sin(theta).*(-8.439375e+2)-sin(theta).^6.*(cos(psi.*5.0).*(1.49e+2./1.0e+1)+sin(psi.*5.0).*(1.09e+2./1.0e+1)).*2.326813808623286+(cos(psi).*(3.19e+2./5.0)-sin(psi).*(9.2e+1./5.0)).*(sqrt(2.1e+1).*cos(theta.*2.0).*(5.0./1.28e+2)+sqrt(2.1e+1).*cos(theta.*4.0).*(3.0./1.6e+1)+sqrt(2.1e+1).*cos(theta.*6.0).*(9.9e+1./1.28e+2))+cos(theta).^3.*sin(theta).*5.063625e+3-cos(theta).^5.*sin(theta).*5.5699875e+3-cos(theta).*sin(theta).^5.*(cos(psi.*6.0).*(3.04e+2./5.0)-sin(psi.*6.0).*(3.64e+2./5.0)).*4.030159736288377+cos(theta).*sin(theta).^5.*(cos(psi.*4.0).*(4.09e+2./1.0e+1)+sin(psi.*4.0).*(2.99e+2./5.0)).*1.091372415814144e+1+cos(theta).^2.*sin(theta).^4.*(cos(psi.*5.0).*(1.49e+2./1.0e+1)+sin(psi.*5.0).*(1.09e+2./1.0e+1)).*1.163406904311643e+1+cos(theta).*sin(theta).^3.*(sin(theta).^2.*1.1e+1-1.0e+1).*(cos(psi.*4.0).*(4.09e+2./1.0e+1)+sin(psi.*4.0).*(2.99e+2./5.0)).*1.984313483298443+(sqrt(2.1e+2).*sin(theta).^4.*(cos(psi.*3.0).*1.157e+2-sin(psi.*3.0).*(4.89e+2./1.0e+1)).*(cos(theta).^2.*1.1e+1-3.0))./1.6e+1-(sqrt(2.1e+2).*sin(theta).^2.*(cos(psi.*2.0).*(7.67e+2./1.0e+1)+sin(psi.*2.0).*(8.4e+1./5.0)).*(cos(theta).*sin(theta).*9.6e+1-cos(theta).*sin(theta).^3.*1.32e+2))./3.2e+1+sqrt(2.1e+2).*cos(theta).^2.*sin(theta).^4.*(cos(psi.*3.0).*1.157e+2-sin(psi.*3.0).*(4.89e+2./1.0e+1)).*(1.1e+1./8.0)+(sqrt(2.1e+2).*cos(theta).*sin(theta).*(cos(psi.*2.0).*(7.67e+2./1.0e+1)+sin(psi.*2.0).*(8.4e+1./5.0)).*(sin(theta).^2.*-4.8e+1+sin(theta).^4.*3.3e+1+1.6e+1))./1.6e+1-sqrt(2.1e+2).*cos(theta).^2.*sin(theta).^2.*(cos(psi.*3.0).*1.157e+2-sin(psi.*3.0).*(4.89e+2./1.0e+1)).*(cos(theta).^2.*1.1e+1-3.0).*(3.0./1.6e+1)).*2.714318712056112e+30+1.0./r.^2.*(sin(theta).*2.935e+4-cos(theta).*(cos(psi).*1.4103e+3-sin(psi).*4.5455e+3)).*2.58596602811e+11-1.0./r.^11.*(cos(theta).*sin(theta).*(-3.519140625e+1)-sin(theta).^10.*(cos(psi.*9.0).*(1.3e+1./5.0)-sin(psi.*9.0).*(9.0./1.0e+1)).*2.65478475211798+cos(theta).^3.*sin(theta).*6.099843749999999e+2-cos(theta).^5.*sin(theta).*2.7449296875e+3+cos(theta).^7.*sin(theta).*4.444171875e+3-cos(theta).^9.*sin(theta).*2.34553515625e+3+cos(theta).*sin(theta).^9.*(cos(psi.*8.0).*(9.0./1.0e+1)-sin(psi.*8.0).*(1.9e+1./5.0)).*1.63651923008246e+1+cos(theta).*sin(theta).^9.*(cos(psi.*1.0e+1).*(3.9e+1./1.0e+1)+sin(psi.*1.0e+1).*9.0).*5.936279171365732+sin(theta).^8.*(cos(psi.*7.0).*(3.0./2.0)-sin(psi.*7.0).*(2.1e+1./5.0)).*(cos(theta).^2.*1.9e+1-3.0).*1.05490449156695-sin(theta).^6.*(cos(psi.*6.0).*(9.0./1.0e+1)-sin(psi.*6.0).*(2.0./5.0)).*(cos(theta).*sin(theta).*1.088e+3-cos(theta).*sin(theta).^3.*1.292e+3).*1.279259601079126e-1-sin(theta).^4.*(cos(psi.*4.0)-sin(psi.*4.0).*(2.7e+1./5.0)).*(cos(theta).*sin(theta).*1.008e+3-cos(theta).*sin(theta).^3.*2.856e+3+cos(theta).*sin(theta).^5.*1.938e+3).*3.618292555284191e-1+sin(theta).^4.*(cos(psi.*3.0).*2.0+sin(psi.*3.0).*(5.0./2.0)).*(cos(theta).^2.*1.05e+2-cos(theta).^4.*3.57e+2+cos(theta).^6.*3.23e+2-7.0).*5.117038404316505e-1+cos(theta).^2.*sin(theta).^8.*(cos(psi.*7.0).*(3.0./2.0)-sin(psi.*7.0).*(2.1e+1./5.0)).*4.008637067954409e+1+cos(theta).^2.*sin(theta).^8.*(cos(psi.*9.0).*(1.3e+1./5.0)-sin(psi.*9.0).*(9.0./1.0e+1)).*2.389306276906182e+1-sin(theta).^6.*(cos(psi.*5.0)./2.0+sin(psi.*5.0).*9.0).*(cos(theta).^2.*-1.7e+2+cos(theta).^4.*3.23e+2+1.5e+1).*2.288409143105751e-1-cos(theta).*sin(theta).^3.*(cos(psi.*4.0)-sin(psi.*4.0).*(2.7e+1./5.0)).*(sin(theta).^2.*5.04e+2-sin(theta).^4.*7.14e+2+sin(theta).^6.*3.23e+2-1.12e+2).*1.447317022113676+cos(theta).*sin(theta).^5.*(cos(psi.*5.0)./2.0+sin(psi.*5.0).*9.0).*(cos(theta).*sin(theta).*3.4e+2-cos(theta).^3.*sin(theta).*1.292e+3).*2.288409143105751e-1+cos(theta).*sin(theta).^7.*(sin(theta).^2.*1.9e+1-1.8e+1).*(cos(psi.*8.0).*(9.0./1.0e+1)-sin(psi.*8.0).*(1.9e+1./5.0)).*3.445303642278863-cos(theta).^2.*sin(theta).^6.*(cos(psi.*7.0).*(3.0./2.0)-sin(psi.*7.0).*(2.1e+1./5.0)).*(cos(theta).^2.*1.9e+1-3.0).*7.384331440968649+sqrt(5.5e+1).*cos(theta).^2.*(cos(psi).*(3.2e+1./5.0)-sin(psi).*(3.3e+1./1.0e+1)).*(cos(theta).^2.*-1.092e+3+cos(theta).^4.*4.914e+3-cos(theta).^6.*7.956e+3+cos(theta).^8.*4.199e+3+6.3e+1).*7.812499999999999e-3+cos(theta).*sin(theta).^3.*(cos(psi.*3.0).*2.0+sin(psi.*3.0).*(5.0./2.0)).*(cos(theta).*sin(theta).*2.1e+2-cos(theta).^3.*sin(theta).*1.428e+3+cos(theta).^5.*sin(theta).*1.938e+3).*5.117038404316505e-1+sqrt(1.65e+2).*sin(theta).^2.*(cos(psi.*2.0)./5.0+sin(psi.*2.0)./1.0e+1).*(cos(theta).*sin(theta).*6.656e+3-cos(theta).*sin(theta).^3.*3.744e+4+cos(theta).*sin(theta).^5.*6.3648e+4-cos(theta).*sin(theta).^7.*3.3592e+4).*3.90625e-3-cos(theta).^2.*sin(theta).^2.*(cos(psi.*3.0).*2.0+sin(psi.*3.0).*(5.0./2.0)).*(cos(theta).^2.*1.05e+2-cos(theta).^4.*3.57e+2+cos(theta).^6.*3.23e+2-7.0).*1.535111521294951-sqrt(5.5e+1).*sin(theta).^2.*(cos(psi).*(3.2e+1./5.0)-sin(psi).*(3.3e+1./1.0e+1)).*(cos(theta).^2.*-1.092e+3+cos(theta).^4.*4.914e+3-cos(theta).^6.*7.956e+3+cos(theta).^8.*4.199e+3+6.3e+1).*7.812499999999999e-3+cos(theta).*sin(theta).^5.*(cos(psi.*6.0).*(9.0./1.0e+1)-sin(psi.*6.0).*(2.0./5.0)).*(sin(theta).^2.*-5.44e+2+sin(theta).^4.*3.23e+2+2.24e+2).*7.675557606474756e-1+cos(theta).^2.*sin(theta).^4.*(cos(psi.*5.0)./2.0+sin(psi.*5.0).*9.0).*(cos(theta).^2.*-1.7e+2+cos(theta).^4.*3.23e+2+1.5e+1).*1.144204571552876-sqrt(1.65e+2).*cos(theta).*sin(theta).*(cos(psi.*2.0)./5.0+sin(psi.*2.0)./1.0e+1).*(sin(theta).^2.*-3.328e+3+sin(theta).^4.*9.36e+3-sin(theta).^6.*1.0608e+4+sin(theta).^8.*4.199e+3+3.84e+2).*7.812499999999999e-3+sqrt(5.5e+1).*cos(theta).*sin(theta).*(cos(psi).*(3.2e+1./5.0)-sin(psi).*(3.3e+1./1.0e+1)).*(cos(theta).*sin(theta).*2.184e+3-cos(theta).^3.*sin(theta).*1.9656e+4+cos(theta).^5.*sin(theta).*4.7736e+4-cos(theta).^7.*sin(theta).*3.3592e+4).*7.812499999999999e-3).*4.471891532119216e+45)./r;
Bpsi = @(psi,r,theta)-(1.0./r.^3.*((sqrt(3.0).*sin(theta).^2.*(cos(psi.*2.0).*1.6284e+3+sin(psi.*2.0).*3.2974e+3))./2.0+(sqrt(3.0).*sin(theta.*2.0).*(cos(psi).*3.1336e+3+sin(psi).*2.9509e+3))./2.0).*-1.647518956508881e+15+1.0./r.^11.*(sin(theta).^10.*(cos(psi.*1.0e+1).*9.0e+1-sin(psi.*1.0e+1).*3.9e+1).*(-5.936279171365732e-1)+cos(theta).*sin(theta).^9.*(cos(psi.*9.0).*(8.1e+1./1.0e+1)+sin(psi.*9.0).*(1.17e+2./5.0)).*2.65478475211798+sin(theta).^8.*(sin(theta).^2.*1.9e+1-1.8e+1).*(cos(psi.*8.0).*(1.52e+2./5.0)+sin(psi.*8.0).*(3.6e+1./5.0)).*4.306629552848578e-1-sin(theta).^4.*(cos(psi.*4.0).*(1.08e+2./5.0)+sin(psi.*4.0).*4.0).*(sin(theta).^2.*5.04e+2-sin(theta).^4.*7.14e+2+sin(theta).^6.*3.23e+2-1.12e+2).*3.618292555284191e-1+sin(theta).^6.*(cos(psi.*6.0).*(1.2e+1./5.0)+sin(psi.*6.0).*(2.7e+1./5.0)).*(sin(theta).^2.*-5.44e+2+sin(theta).^4.*3.23e+2+2.24e+2).*1.279259601079126e-1-cos(theta).*sin(theta).^7.*(cos(psi.*7.0).*(1.47e+2./5.0)+sin(psi.*7.0).*(2.1e+1./2.0)).*(cos(theta).^2.*1.9e+1-3.0).*1.05490449156695+cos(theta).*sin(theta).^3.*(cos(psi.*3.0).*(1.5e+1./2.0)-sin(psi.*3.0).*6.0).*(cos(theta).^2.*1.05e+2-cos(theta).^4.*3.57e+2+cos(theta).^6.*3.23e+2-7.0).*5.117038404316505e-1+sqrt(1.65e+2).*sin(theta).^2.*(cos(psi.*2.0)./5.0-sin(psi.*2.0).*(2.0./5.0)).*(sin(theta).^2.*-3.328e+3+sin(theta).^4.*9.36e+3-sin(theta).^6.*1.0608e+4+sin(theta).^8.*4.199e+3+3.84e+2).*3.90625e-3-cos(theta).*sin(theta).^5.*(cos(psi.*5.0).*4.5e+1-sin(psi.*5.0).*(5.0./2.0)).*(cos(theta).^2.*-1.7e+2+cos(theta).^4.*3.23e+2+1.5e+1).*2.288409143105751e-1+sqrt(5.5e+1).*cos(theta).*sin(theta).*(cos(psi).*(3.3e+1./1.0e+1)+sin(psi).*(3.2e+1./5.0)).*(cos(theta).^2.*-1.092e+3+cos(theta).^4.*4.914e+3-cos(theta).^6.*7.956e+3+cos(theta).^8.*4.199e+3+6.3e+1).*7.812499999999999e-3).*4.471891532119216e+45+1.0./r.^7.*(sin(theta).^6.*(cos(psi.*6.0).*4.368e+2+sin(psi.*6.0).*3.648e+2).*6.716932893813961e-1-(cos(psi).*(9.2e+1./5.0)+sin(psi).*(3.19e+2./5.0)).*(sqrt(2.1e+1).*sin(theta.*2.0).*(5.0./2.56e+2)+sqrt(2.1e+1).*sin(theta.*4.0).*(3.0./6.4e+1)+sqrt(2.1e+1).*sin(theta.*6.0).*(3.3e+1./2.56e+2))+cos(theta).*sin(theta).^5.*(cos(psi.*5.0).*(1.09e+2./2.0)-sin(psi.*5.0).*(1.49e+2./2.0)).*2.326813808623286+sin(theta).^4.*(sin(theta).^2.*1.1e+1-1.0e+1).*(cos(psi.*4.0).*2.392e+2-sin(psi.*4.0).*(8.18e+2./5.0)).*4.960783708246107e-1+(sqrt(2.1e+2).*sin(theta).^2.*(cos(psi.*2.0).*(1.68e+2./5.0)-sin(psi.*2.0).*(7.67e+2./5.0)).*(sin(theta).^2.*-4.8e+1+sin(theta).^4.*3.3e+1+1.6e+1))./3.2e+1+(sqrt(2.1e+2).*cos(theta).*sin(theta).^3.*(cos(psi.*3.0).*1.467e+2+sin(psi.*3.0).*3.471e+2).*(cos(theta).^2.*1.1e+1-3.0))./1.6e+1).*2.714318712056112e+30-1.0./r.^4.*((sqrt(1.0e+1).*sin(theta).^3.*(cos(psi.*3.0).*1.6488e+3+sin(psi.*3.0).*1.3602e+3))./4.0-(sqrt(6.0).*sin(theta).*(sin(theta).^2.*5.0-4.0).*(cos(psi).*(5.69e+2./1.0e+1)-sin(psi).*2.4042e+3))./4.0+(sqrt(1.5e+1).*cos(theta).*(cos(psi.*2.0).*4.752e+2-sin(psi.*2.0).*2.4876e+3).*(cos(theta).^2-1.0))./2.0).*1.049634327191808e+19+1.0./r.^8.*(sin(theta).^7.*(cos(psi.*7.0).*(7.7e+1./5.0)+sin(psi.*7.0).*1.001e+2).*(-6.472598492877493e-1)-cos(theta).*sin(theta).^6.*(cos(psi.*6.0).*(7.53e+2./5.0)-sin(psi.*6.0).*(3.36e+2./5.0)).*2.421824596249695+sin(theta).^5.*(sin(theta).^2.*1.3e+1-1.2e+1).*(cos(psi.*5.0).*3.7e+1+sin(psi.*5.0).*(2.5e+1./2.0)).*4.749588797990833e-1+cos(theta).*sin(theta).^4.*(cos(psi.*4.0).*9.4e+1-sin(psi.*4.0).*(3.16e+2./5.0)).*(cos(theta).^2.*1.3e+1-3.0).*9.499177595981665e-1-sqrt(2.1e+1).*sin(theta).^3.*(cos(psi.*3.0).*3.0+sin(psi.*3.0).*1.779e+2).*(sin(theta).^2.*-2.2e+2+sin(theta).^4.*1.43e+2+8.0e+1).*3.125e-2+sqrt(4.2e+1).*cos(theta).*(cos(psi.*2.0).*(1.44e+2./5.0)-sin(psi.*2.0).*(8.8e+1./5.0)).*(cos(theta).^2.*1.25e+2-cos(theta).^4.*2.53e+2+cos(theta).^6.*1.43e+2-1.5e+1).*3.125e-2+sqrt(7.0).*sin(theta).*(cos(psi).*(4.89e+2./1.0e+1)-sin(psi).*(7.69e+2./1.0e+1)).*(sin(theta).^2.*4.32e+2-sin(theta).^4.*7.92e+2+sin(theta).^6.*4.29e+2-6.4e+1).*3.125e-2).*1.729292451450949e+34+1.0./r.^9.*((cos(psi).*(3.6e+1./5.0)-sin(psi).*(1.09e+2./1.0e+1)).*(sin(theta.*2.0).*5.126953125e-2+sin(theta.*4.0).*1.1279296875e-1+sin(theta.*6.0).*2.0947265625e-1+sin(theta.*8.0).*5.23681640625e-1)+sin(theta).^8.*(cos(psi.*8.0).*(1.56e+2./5.0)-sin(psi.*8.0).*8.0).*6.267066542400439e-1-cos(theta).*sin(theta).^7.*(cos(psi.*7.0).*(1.82e+2./5.0)-sin(psi.*7.0).*(5.88e+2./5.0)).*2.506826616960176-sin(theta).^6.*(sin(theta).^2.*1.5e+1-1.4e+1).*(cos(psi.*6.0).*(2.1e+1./5.0)-sin(psi.*6.0).*(4.47e+2./5.0)).*4.576818286211503e-1-sin(theta).^4.*(cos(psi.*4.0).*(1.94e+2./5.0)-sin(psi.*4.0).*(4.36e+2./5.0)).*(sin(theta).^2.*-1.04e+2+sin(theta).^4.*6.5e+1+4.0e+1).*4.113264556590057e-1+cos(theta).*sin(theta).^5.*(cos(psi.*5.0).*(1.27e+2./2.0)-sin(psi.*5.0).*(1.69e+2./2.0)).*(cos(theta).^2.*5.0-1.0).*2.96611725366682+cos(theta).*sin(theta).^3.*(cos(psi.*3.0).*(6.9e+1./2.0)-sin(psi.*3.0).*6.0).*(cos(theta).^2.*-2.6e+1+cos(theta).^4.*3.9e+1+3.0).*1.062040341747902+sqrt(7.0e+1).*sin(theta).^2.*(cos(psi.*2.0).*(1.26e+2./5.0)-sin(psi.*2.0).*3.5e+1).*(sin(theta).^2.*1.76e+2-sin(theta).^4.*2.86e+2+sin(theta).^6.*1.43e+2-3.2e+1).*4.6875e-2).*1.1017322208194e+38-1.0./r.^10.*(sin(theta).^9.*(cos(psi.*9.0).*(4.41e+2./5.0)+sin(psi.*9.0).*(5.76e+2./5.0)).*(-6.090493921755238e-1)-cos(theta).*sin(theta).^8.*(cos(psi.*8.0).*(3.2e+1./5.0)+sin(psi.*8.0).*(3.48e+2./5.0)).*2.583977731709148-sin(theta).^7.*(sin(theta).^2.*1.7e+1-1.6e+1).*(cos(psi.*7.0).*(2.1e+1./5.0)+sin(psi.*7.0).*(3.01e+2./5.0)).*4.431485250278681e-1+sin(theta).^3.*(cos(psi.*3.0).*(2.49e+2./1.0e+1)+sin(psi.*3.0).*(3.0./5.0)).*(sin(theta).^2.*3.12e+2-sin(theta).^4.*4.68e+2+sin(theta).^6.*2.21e+2-6.4e+1).*3.754879637718099e-1+sin(theta).^5.*(cos(psi.*5.0).*(5.3e+1./2.0)-sin(psi.*5.0).*(1.31e+2./2.0)).*(sin(theta).^2.*-1.4e+2+sin(theta).^4.*8.5e+1+5.6e+1).*3.96364090436432e-1-cos(theta).*sin(theta).^6.*(cos(psi.*6.0).*(2.16e+2./5.0)-sin(psi.*6.0).*(7.2e+1./5.0)).*(cos(theta).^2.*1.7e+1-3.0).*1.023407680863301+sqrt(5.0).*sin(theta).*(cos(psi).*(1.24e+2./5.0)+sin(psi).*8.0).*(sin(theta).^2.*-1.408e+3+sin(theta).^4.*4.576e+3-sin(theta).^6.*5.72e+3+sin(theta).^8.*2.431e+3+1.28e+2).*2.34375e-2+cos(theta).*sin(theta).^4.*(cos(psi.*4.0).*(6.8e+1./5.0)-sin(psi.*4.0).*1.0e+1).*(cos(theta).^2.*-1.0e+1+cos(theta).^4.*1.7e+1+1.0).*3.316219904216999+sqrt(1.1e+2).*cos(theta).*(cos(psi.*2.0).*(1.21e+2./5.0)-sin(psi.*2.0).*6.0).*(cos(theta).^2.*-9.8e+1+cos(theta).^4.*3.64e+2-cos(theta).^6.*4.94e+2+cos(theta).^8.*2.21e+2+7.0).*4.6875e-2).*7.019135978840395e+41+1.0./r.^5.*(((sqrt(1.0e+1).*sin(theta.*2.0))./1.6e+1+sqrt(1.0e+1).*sin(theta.*4.0).*(7.0./3.2e+1)).*(cos(psi).*2.786e+2-sin(psi).*7.996e+2)-(sqrt(3.5e+1).*sin(theta).^4.*(cos(psi.*4.0).*1.5016e+3+sin(psi.*4.0).*4.8e+1))./8.0+(sqrt(7.0e+1).*cos(theta).*sin(theta).^3.*(cos(psi.*3.0).*6.36e+2+sin(psi.*3.0).*8.433e+2))./4.0+(sqrt(5.0).*sin(theta).^2.*(sin(theta).^2.*7.0-6.0).*(cos(psi.*2.0).*2.68e+2+sin(psi.*2.0).*(5.58e+2./5.0)))./4.0).*6.687220298539009e+22+1.0./r.^6.*(sin(theta).^5.*(cos(psi.*5.0).*5.31e+2-sin(psi.*5.0).*(2.09e+2./2.0)).*7.01560760020114e-1+cos(theta).*sin(theta).^4.*(cos(psi.*4.0).*(8.58e+2./5.0)+sin(psi.*4.0).*5.676e+2).*2.218529918662356+sqrt(1.5e+1).*(cos(psi).*(4.53e+2./1.0e+1)-sin(psi).*3.69e+2).*(sin(theta)-sin(theta).^3.*(7.0./2.0)+sin(theta).^5.*(2.1e+1./8.0))+(sqrt(7.0e+1).*sin(theta).^3.*(sin(theta).^2.*9.0-8.0).*(cos(psi.*3.0).*3.687e+2-sin(psi.*3.0).*4.161e+2))./1.6e+1-(sqrt(1.05e+2).*cos(theta).*(cos(psi.*2.0).*4.4e+2-sin(psi.*2.0).*3.744e+2).*(cos(theta).^2.*-4.0+cos(theta).^4.*3.0+1.0))./4.0).*4.260428052199203e+26+1.0./r.^2.*sin(theta).*(cos(psi).*4.5455e+3+sin(psi).*1.4103e+3).*2.58596602811e+11)./(r.*sin(theta));

%%
long = alfa - alfa_G; % Longitude of the spacecraft
lat = delta; % Latitude of the spacecraft
colat = pi/2 - delta; % Colatitude of the spacecraft
Br = Br(long, r_scalar, colat);
Btheta = Btheta(long, r_scalar, colat);
Bpsi = Bpsi(long, r_scalar, colat);



%% Components of B wrt the inertial frame
B_IN=zeros(3,1);


B_IN(1,1) =  (Br*cos(lat) + Btheta*sin(lat))*cos(alfa) - Bpsi*sin(alfa);
B_IN(2,1) =  (Br*cos(lat) + Btheta*sin(lat))*sin(alfa) + Bpsi*cos(alfa);
B_IN(3,1) =  (Br*sin(lat) - Btheta*cos(lat));
B_IN = B_IN*10^-9;
